simulink library "test"  (R2023a)
settings: Solver=VariableStepAuto  StartTime=0.0  StopTime=10.0  RelTol=1e-3
settings Model: Creator=Qw011  LastModifiedBy=Qw011

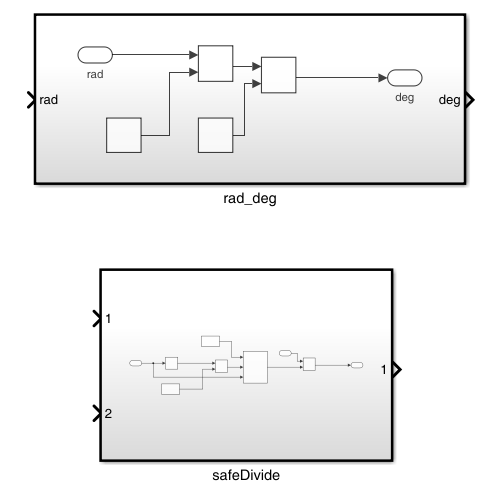
[thumbnail: Simulink's stored preview of the top-level diagram]
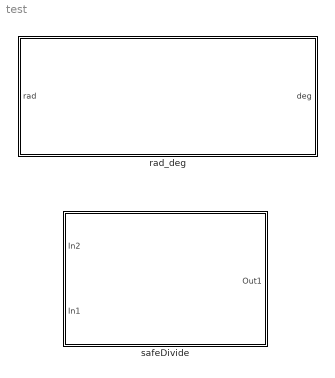
== system test ==
  rad_deg : Subsystem  TreatAsAtomicUnit=on
      settings: RTWFcnNameOpts=Use subsystem name
  safeDivide : Subsystem  TreatAsAtomicUnit=on
      settings: RTWFcnNameOpts=Use subsystem name

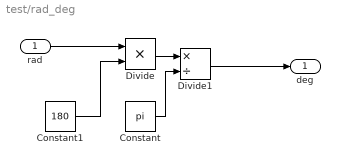
== system test/rad_deg ==
  rad : Inport
  Constant : Constant  Value=pi
  Constant1 : Constant  Value=180
  Divide : Product  Inputs=**
  Divide1 : Product  Inputs=*/
  deg : Outport
  wires:
  rad/1 -> Divide/1
  Constant1/1 -> Divide/2
  Divide/1 -> Divide1/1
  Constant/1 -> Divide1/2
  Divide1/1 -> deg/1

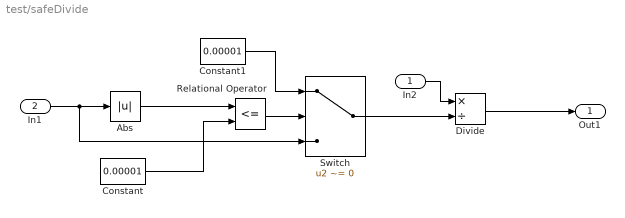
== system test/safeDivide ==
  In2 : Inport
  In1 : Inport  Port=2
  Abs : Abs  SaturateOnIntegerOverflow=off
  Constant : Constant  Value=0.00001
  Constant1 : Constant  Value=0.00001
  Divide : Product  Inputs=*/
  Relational Operator : RelationalOperator  Operator=<=  OutDataTypeStr=boolean  RndMeth=Simplest  InputSameDT=off
  Switch : Switch  Criteria=u2 ~= 0  SaturateOnIntegerOverflow=off  InputSameDT=off
  Out1 : Outport
  wires:
  In1/1 -> Switch/3, Abs/1
  Abs/1 -> Relational Operator/1
  Constant/1 -> Relational Operator/2
  Relational Operator/1 -> Switch/2
  Constant1/1 -> Switch/1
  Divide/1 -> Out1/1
  In2/1 -> Divide/1
  Switch/1 -> Divide/2
